simulink model "backflowblocks_test"  (R2024b)
settings: Solver=FixedStepDiscrete  StartTime=0.0  StopTime=5  FixedStep=0.0002  RelTol=1e-3
InitFcn:
  |    parameters_charlton;
  |    parameters_ferreira;
  |    parameters_backflowcontrol;
undefined symbols (not defined in the file): H_REF_MAX, H_REF_MIN, HR, Ki_fb, Kp_fb, LUT_Q, LUT_u, N, Ts, U_FB_MAX
libraries: slpidlib x1, simulink x1
settings Model: Creator=sammy  LastModifiedBy=sammy

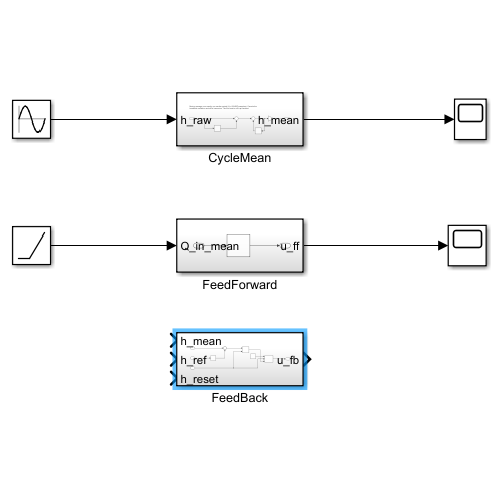
[thumbnail: Simulink's stored preview of the top-level diagram]
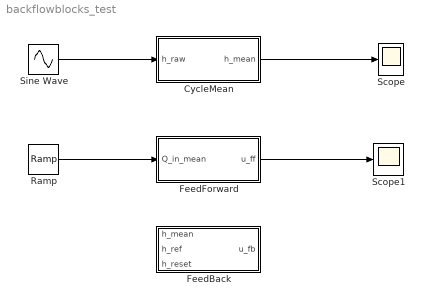
== system backflowblocks_test ==
  CycleMean : Subsystem
  FeedBack : Subsystem
  FeedForward : Subsystem
  Ramp : simulink/Sources/Ramp  slope=10  start=0  InitialOutput=0
  Scope : Scope
  Scope1 : Scope
  Sine Wave : Sin  Amplitude=10  Frequency=2*pi*HR/60  SampleTime=0
  wires:
  Sine Wave/1 -> CycleMean/1(h_raw)
  CycleMean/1(h_mean) -> Scope/1
  Ramp/1 -> FeedForward/1(Q_in_mean)
  FeedForward/1(u_ff) -> Scope1/1

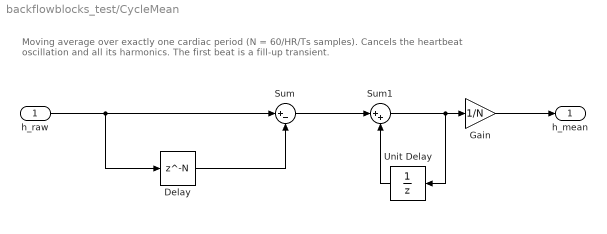
== system backflowblocks_test/CycleMean ==
  note: Moving average over exactly one cardiac period (N = 60/HR/Ts samples). Cancels the heartbeat oscillation and all its harmonics. The first beat is a fill-up transient.
  h_raw : Inport
  Delay : Delay  DelayLength=N
  Gain : Gain  Gain=1/N
  Sum : Sum  Inputs=|+-
  Sum1 : Sum  Inputs=|++
  Unit Delay : UnitDelay  SampleTime=-1  HasFrameUpgradeWarning=on
  h_mean : Outport
  wires:
  h_raw/1 -> Sum/1, Delay/1
  Delay/1 -> Sum/2
  Sum/1 -> Sum1/1
  Sum1/1 -> Unit Delay/1, Gain/1
  Gain/1 -> h_mean/1
  Unit Delay/1 -> Sum1/2

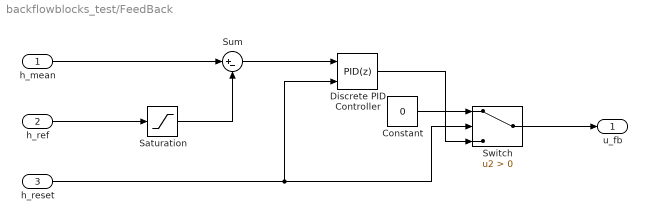
== system backflowblocks_test/FeedBack ==
  h_mean : Inport  SampleTime=Ts
  h_ref : Inport  Port=2  SampleTime=Ts
  h_reset : Inport  Port=3  SampleTime=Ts
  Constant : Constant  Value=0
  Discrete PID Controller : slpidlib/PID Controller  Controller=PID  Form=Parallel  TimeDomain=Discrete-time  UseExternalTs=off  SampleTime=Ts  IntegratorMethod=Forward Euler  FilterMethod=Forward Euler  ControllerParametersSource=internal  P=Kp_fb  I=Ki_fb  UseKiTs=off  D=0  UseExternalDerivativeSource=off  N=100  UseFilter=on  TunerSelectOption=Transfer Function Based (PID Tuner App)  InitialConditionSource=internal  InitialConditionForIntegrator=0  InitialConditionForFilter=0  DifferentiatorICPrevScaledInput=0  ExternalReset=level  TrackingMode=off  Kt=1  LimitOutput=on  SatLimitsSource=internal  UpperSaturationLimit=U_FB_MAX  LowerSaturationLimit=-U_FB_MAX  LinearizeAsGain=off  AntiWindupMode=clamping  Kb=1  LimitIntegrator=off  UpperIntegratorSaturationLimit=inf  LowerIntegratorSaturationLimit=-inf  POutMin=[]  POutMax=[]  IOutMin=[]  IOutMax=[]  DOutMin=[]  DOutMax=[]  NOutMin=[]  NOutMax=[]  SumOutMin=[]  SumOutMax=[]  SaturationOutMin=[]  SaturationOutMax=[]  PParamMin=[]  PParamMax=[]  IParamMin=[]  IParamMax=[]  DParamMin=[]  DParamMax=[]  NParamMin=[]  NParamMax=[]  KbParamMin=[]  KbParamMax=[]  KtParamMin=[]  KtParamMax=[]  KbOutMin=[]  KbOutMax=[]  KtOutMin=[]  KtOutMax=[]  IntegratorOutMin=[]  IntegratorOutMax=[]  FilterOutMin=[]  FilterOutMax=[]  SumI1OutMin=[]  SumI1OutMax=[]  SumI2OutMin=[]  SumI2OutMax=[]  SumI3OutMin=[]  SumI3OutMax=[]  SumI4OutMin=[]  SumI4OutMax=[]  SumDOutMin=[]  SumDOutMax=[]  DifferentiatorOutMin=[]  DifferentiatorOutMax=[]  FilterDiffOutCoefMin=[]  FilterDiffOutCoefMax=[]  ReciprocalOutMin=[]  ReciprocalOutMax=[]  SumDenOutMin=[]  SumDenOutMax=[]  SumNumOutMin=[]  SumNumOutMax=[]  DivideOutMin=[]  DivideOutMax=[]  UdiffTsProdOutMin=[]  UdiffTsProdOutMax=[]  NTsProdOutMin=[]  NTsProdOutMax=[]  UintegralTsProdOutMin=[]  UintegralTsProdOutMax=[]  UngainTsProdOutMin=[]  UngainTsProdOutMax=[]  ClampingZeroOutDataTypeStr=Inherit: Inherit via back propagation  ClampingZeroOutMin=[]  ClampingZeroOutMax=[]  FilterDenConstantOutDataTypeStr=Inherit: Inherit via back propagation  FilterDenConstantOutMin=[]  FilterDenConstantOutMax=[]  PCopyOutDataTypeStr=Inherit: Inherit via back propagation  PCopyOutMin=[]  PCopyOutMax=[]  NCopyOutDataTypeStr=Inherit: Inherit via back propagation  NCopyOutMin=[]  NCopyOutMax=[]  IntegratorContinuousStateAttributes=''  IntegratorStateMustResolveToSignalObject=off  IntegratorRTWStateStorageClass=Auto  FilterContinuousStateAttributes=''  FilterStateMustResolveToSignalObject=off  FilterRTWStateStorageClass=Auto  ParallelPVariant=InternalParameters  IdealPVariant=Disabled  IVariant=InternalParameters  DVariant=InternalParameters  IntegratorVariant=Discrete  SatVariant=Enabled  AWVariant=DiscClampingParallel  PCopyVariant=Disabled  TRVariant=Disabled  FdbkBlocksVariant=Forward  IdealPFdbkVariant=Disabled  SatFdbkVariant=Disabled  DerivativeFilterVariant=ForwardEulerFilter  NVariant=InternalParameters  NCopyVariant=Disabled  FilterICVariant=InternalICsFilter  IntegratorICVariant=InternalICs  ExternalResetVariant=ExternalReset  TRSumVariant=Passthrough  SumFdbkVariant=Disabled  SumVariant=Sum_PID  TsampFilterVariant=InternalTs  TsampNgainVariant=Passthrough  TsampIntegralVariant=Disabled_SignalSpec  ExternalSaturationOutDataTypeStr=Inherit: Same as second input  DerivativeSourceVariant=ErrorSignal  PreIntVariant=InternalPreInt
      settings: LibrarySourceBlock=simulink/Discrete/Discrete PID Controller
  Saturation : Saturate  UpperLimit=H_REF_MAX  LowerLimit=H_REF_MIN
  Sum : Sum  Inputs=|+-
  Switch : Switch  Criteria=u2 > Threshold  SaturateOnIntegerOverflow=off  InputSameDT=off
  u_fb : Outport
  wires:
  h_ref/1 -> Saturation/1
  Saturation/1 -> Sum/2
  h_mean/1 -> Sum/1
  Sum/1 -> Discrete PID Controller/1
  h_reset/1 -> Switch/2, Discrete PID Controller/2
  Discrete PID Controller/1 -> Switch/3
  Constant/1 -> Switch/1
  Switch/1 -> u_fb/1

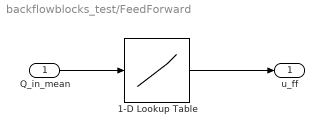
== system backflowblocks_test/FeedForward ==
  Q_in_mean : Inport  SampleTime=Ts
  1-D Lookup Table : Lookup_n-D  NumberOfTableDimensions=1  BreakpointsForDimension1=LUT_Q  Table=LUT_u  InterpMethod=Linear Lagrange  ExtrapMethod=Clip  InternalRulePriority=Speed  RndMeth=Simplest
  u_ff : Outport
  wires:
  Q_in_mean/1 -> 1-D Lookup Table/1
  1-D Lookup Table/1 -> u_ff/1
